simulink model "inverted_pendulum_mpc"  (R2025a)
settings: Solver=ode45  StartTime=0.0  StopTime=30  MaxStep=0.01  RelTol=1e-3
model workspace (MAT data in the model file):
  disturbance_signal = [0  0; 30.1  0]
  mpc_controller = mpc
  mpc_controller.Ts = 0.05
  mpc_controller.PredictionHorizon = 50
  mpc_controller.ControlHorizon = 10
  mpc_controller.Model.Plant = ss
  mpc_controller.Model.Plant.InputName_ = "MV1"
  mpc_controller.Model.Plant.InputGroup_.Manipulated = 1
  mpc_controller.Model.Plant.OutputName_ = ["MO1"; "MO2"; "MO3"; "MO4"]
  mpc_controller.Model.Plant.OutputGroup_.Measured = [1 2 3 4]
  mpc_controller.Model.Plant.IOSize_ = [4 1]
  mpc_controller.Model.Plant.Data_ = ltipack.ssdata
  mpc_controller.Model.Plant.Data_.a = [0  1  0  0; 0  0  -2.4525  0.005; 0  0  0  1; 0  0  12.2625  -0.025]
  mpc_controller.Model.Plant.Data_.b = [0; 0.5; 0; -0.5]
  mpc_controller.Model.Plant.Data_.c = [1  0  0  0; 0  1  0  0; 0  0  1  0; 0  0  0  1]
  mpc_controller.Model.Plant.Data_.d = [0; 0; 0; 0]
  mpc_controller.Model.Plant.Data_.dx0 = [0; 0; 0; 0]
  mpc_controller.Model.Plant.Data_.x0 = [0; 0; 0; 0]
  mpc_controller.Model.Plant.Data_.u0 = 0
  mpc_controller.Model.Plant.Data_.y0 = [0; 0; 0; 0]
  mpc_controller.Model.Plant.Data_.Delay.Input = 0
  mpc_controller.Model.Plant.Data_.Delay.Output = [0; 0; 0; 0]
  mpc_controller.Model.Plant.Data_.Delay.Internal = []
  mpc_controller.Model.Plant.Data_.Ts = 0
  mpc_controller.Model.Disturbance = []
  mpc_controller.Model.Noise = []
  mpc_controller.Model.Nominal.X = [0; 0; 0; 0]
  mpc_controller.Model.Nominal.DX = [0; 0; 0; 0]
  mpc_controller.Model.Nominal.U = 0
  mpc_controller.Model.Nominal.Y = [0; 0; 0; 0]
  mpc_controller.ManipulatedVariables.Min = -10
  mpc_controller.ManipulatedVariables.Max = 10
  mpc_controller.ManipulatedVariables.MinECR = 0
  mpc_controller.ManipulatedVariables.MaxECR = 0
  mpc_controller.ManipulatedVariables.RateMin = -Inf
  mpc_controller.ManipulatedVariables.RateMax = Inf
  mpc_controller.ManipulatedVariables.RateMinECR = 0
  mpc_controller.ManipulatedVariables.RateMaxECR = 0
  mpc_controller.ManipulatedVariables.Target = 'nominal'
  mpc_controller.ManipulatedVariables.Name = 'MV1'
  mpc_controller.ManipulatedVariables.Units = ''
  mpc_controller.ManipulatedVariables.ScaleFactor = 1
  mpc_controller.ManipulatedVariables.Type = 'continuous'
  mpc_controller.OutputVariables(1).Min = -Inf
  mpc_controller.OutputVariables(1).Max = Inf
  mpc_controller.OutputVariables(1).MinECR = 1
  mpc_controller.OutputVariables(1).MaxECR = 1
  mpc_controller.OutputVariables(1).Name = 'MO1'
  mpc_controller.OutputVariables(1).Units = ''
  mpc_controller.OutputVariables(1).ScaleFactor = 1
  mpc_controller.OutputVariables(2).Min = -Inf
  mpc_controller.OutputVariables(2).Max = Inf
  mpc_controller.OutputVariables(2).MinECR = 1
  mpc_controller.OutputVariables(2).MaxECR = 1
  mpc_controller.OutputVariables(2).Name = 'MO2'
  mpc_controller.OutputVariables(2).Units = ''
  mpc_controller.OutputVariables(2).ScaleFactor = 1
  mpc_controller.OutputVariables(3).Min = -Inf
  mpc_controller.OutputVariables(3).Max = Inf
  mpc_controller.OutputVariables(3).MinECR = 1
  mpc_controller.OutputVariables(3).MaxECR = 1
  mpc_controller.OutputVariables(3).Name = 'MO3'
  mpc_controller.OutputVariables(3).Units = ''
  mpc_controller.OutputVariables(3).ScaleFactor = 1
  mpc_controller.OutputVariables(4).Min = -Inf
  mpc_controller.OutputVariables(4).Max = Inf
  mpc_controller.OutputVariables(4).MinECR = 1
  mpc_controller.OutputVariables(4).MaxECR = 1
  mpc_controller.OutputVariables(4).Name = 'MO4'
  mpc_controller.OutputVariables(4).Units = ''
  mpc_controller.OutputVariables(4).ScaleFactor = 1
  mpc_controller.Weights.ManipulatedVariables = 0.707106781187
  mpc_controller.Weights.ManipulatedVariablesRate = 0.1
  mpc_controller.Weights.OutputVariables = [2 1.41421356237 17.3205080757 3.16227766017]
  mpc_controller.Weights.ECR = 100000
  mpc_controller.Optimizer.OptimizationType = 'QP'
  mpc_controller.Optimizer.Solver = 'active-set'
  mpc_controller.Optimizer.SolverOptions = mpc.solver.options.qp.ActiveSet
  mpc_controller.Optimizer.SolverOptions.SolverName = 'ActiveSet'
  mpc_controller.Optimizer.MinOutputECR = 0
  mpc_controller.Optimizer.UseSuboptimalSolution = 0
  mpc_controller.Optimizer.CustomSolver = 0
  mpc_controller.Optimizer.CustomSolverCodeGen = 0
  mpc_controller.History = [2026 11 2 14 24 58.008164]
  mpc_controller.MPCData = mpcdata
  mpc_controller.MPCData.IsDirty = 1
  mpc_controller.MPCData.Ts = 0.05
  mpc_controller.MPCData.p = 50
  mpc_controller.MPCData.m = 10
  mpc_controller.MPCData.UseActiveSetSolver = 1
  mpc_controller.MPCData.UseSuboptimalSolution = 0
  mpc_controller.MPCData.CustomSolver = 0
  mpc_controller.MPCData.CustomSolverCodeGen = 0
  mpc_controller.MPCData.IsCustomEstimation = 1
  mpc_controller.MPCData.Uscale = 1
  mpc_controller.MPCData.Yscale = [1; 1; 1; 1]
  mpc_controller.MPCData.mvindex = 1
  mpc_controller.MPCData.myindex = [1; 2; 3; 4]
  mpc_controller.IsEmpty = 0
  mpc_controller.OldOVIntegrator = {[]; []; []; []}
  mpc_controller.EstGain = 'custom'
  mpc_controller.OutDistModel = ss
  mpc_controller.OutDistModel.IOSize_ = [4 1]
  mpc_controller.OutDistModel.Data_ = ltipack.ssdata
  mpc_controller.OutDistModel.Data_.d = [0; 0; 0; 0]
  mpc_controller.OutDistModel.Data_.u0 = 0
  mpc_controller.OutDistModel.Data_.y0 = [0; 0; 0; 0]
  mpc_controller.OutDistModel.Data_.Delay.Input = 0
  mpc_controller.OutDistModel.Data_.Delay.Output = [0; 0; 0; 0]
  mpc_controller.OutDistModel.Data_.Delay.Internal = []
  mpc_controller.OutDistModel.Data_.Ts = 0
  mpc_controller.Version = '25.1'
libraries: mpclib x1
settings Model: Creator=user  LastModifiedBy=user
settings DataIOCC: SaveOutput=off  SaveTime=off

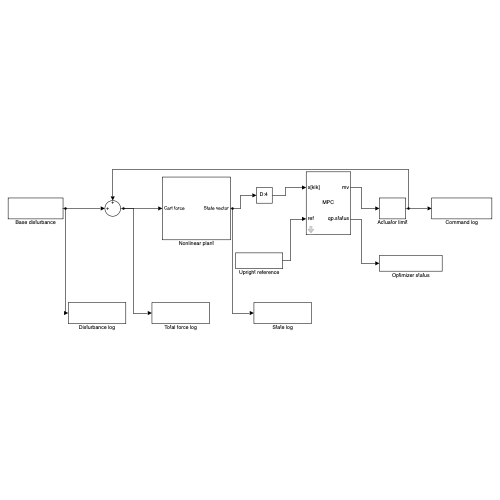
[thumbnail: Simulink's stored preview of the top-level diagram]
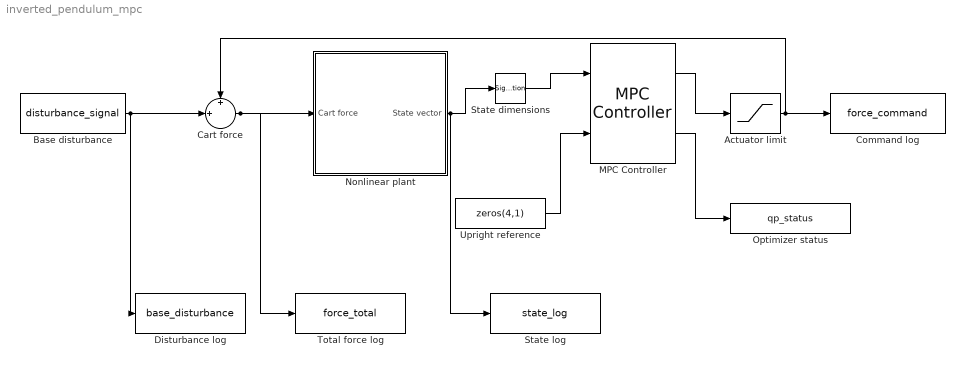
== system inverted_pendulum_mpc ==
  Actuator limit : Saturate  UpperLimit=10  LowerLimit=-10
  Base disturbance : FromWorkspace  VariableName=disturbance_signal  Interpolate=off  OutputAfterFinalValue=Holding final value
  Cart force : Sum  Inputs=+|+||
  Command log : ToWorkspace  VariableName=force_command  SaveFormat=Timeseries  SampleTime=-1
  Disturbance log : ToWorkspace  VariableName=base_disturbance  SaveFormat=Timeseries  SampleTime=-1
  MPC Controller : mpclib/MPC Controller  SCDEnableBlockLinearizationSpecification=on  mpcobj=mpc_controller  is_multiple=0  enable_value=0  return_u0=off  updateMPCinCallerWorkspace=on  md_inport=off  mv_inport=off  uref_inport=off  return_cost=off  return_mvseq=off  return_qpstatus=on  return_xseq=off  return_state=off  return_ovseq=off  state_inport=on  umin_inport=off  umax_inport=off  ymin_inport=off  ymax_inport=off  cc_inport=off  ywt_inport=off  uwt_inport=off  duwt_inport=off  rhoeps_inport=off  pm_inport=off  MaximumP=10  HorizonChoice=FixedHorizon  n_ts=1  n_p=10  n_mv=1  n_md=1  n_ud=0  n_mo=1  n_uo=0  BlockDataType=double  SampleTimeInherited=off  switch_inport=off
  Nonlinear plant : Subsystem
  Optimizer status : ToWorkspace  VariableName=qp_status  SaveFormat=Timeseries  SampleTime=-1
  State dimensions : SignalSpecification  Dimensions=4
  State log : ToWorkspace  VariableName=state_log  SaveFormat=Timeseries  SampleTime=-1
  Total force log : ToWorkspace  VariableName=force_total  SaveFormat=Timeseries  SampleTime=-1
  Upright reference : Constant  Value=zeros(4,1)
  wires:
  Base disturbance/1 -> Cart force/2, Disturbance log/1
  Cart force/1 -> Nonlinear plant/1(Cart force), Total force log/1
  Nonlinear plant/1(State vector) -> State dimensions/1, State log/1
  State dimensions/1 -> MPC Controller/1
  Upright reference/1 -> MPC Controller/2
  MPC Controller/1 -> Actuator limit/1
  MPC Controller/2 -> Optimizer status/1
  Actuator limit/1 -> Cart force/1, Command log/1

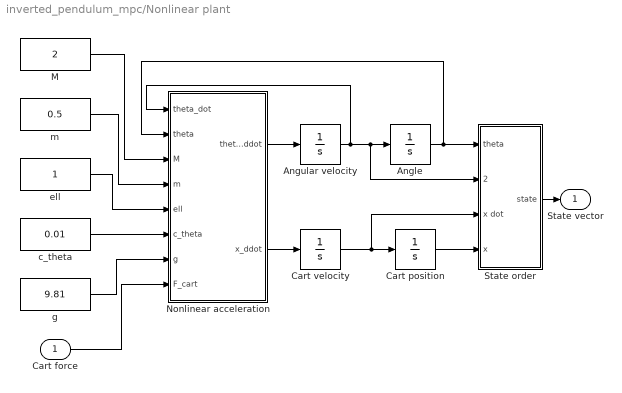
== system inverted_pendulum_mpc/Nonlinear plant ==
  Cart force : Inport
  Angle : Integrator  InitialCondition=5*pi/180
  Angular velocity : Integrator
  Cart position : Integrator
  Cart velocity : Integrator
  M : Constant  Value=2
  Nonlinear acceleration : MATLAB Function  TreatAsAtomicUnit=on
  State order : Subsystem
      mask Display: port_label('input',1,'theta');port_label('input',2,'theta dot');port_label('input',3,'x dot');port_label('input',4,'x');port_label('output',1,'state');
  c_theta : Constant  Value=0.01
  ell : Constant
  g : Constant  Value=9.81
  m : Constant  Value=0.5
  State vector : Outport
  wires:
  M/1 -> Nonlinear acceleration/3(M)
  m/1 -> Nonlinear acceleration/4(m)
  ell/1 -> Nonlinear acceleration/5(ell)
  c_theta/1 -> Nonlinear acceleration/6(c_theta)
  g/1 -> Nonlinear acceleration/7(g)
  Cart force/1 -> Nonlinear acceleration/8(F_cart)
  Nonlinear acceleration/1(theta_ddot) -> Angular velocity/1
  Nonlinear acceleration/2(x_ddot) -> Cart velocity/1
  Angular velocity/1 -> Angle/1, State order/2(theta dot), Nonlinear acceleration/1(theta_dot)
  Cart velocity/1 -> Cart position/1, State order/3(x dot)
  Angle/1 -> Nonlinear acceleration/2(theta), State order/1(theta)
  Cart position/1 -> State order/4(x)
  State order/1(state) -> State vector/1

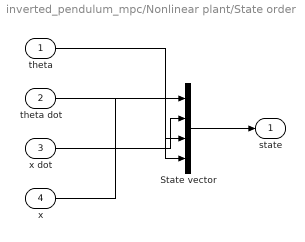
== system inverted_pendulum_mpc/Nonlinear plant/State order ==
  theta : Inport
  theta dot : Inport  Port=2
  x dot : Inport  Port=3
  x : Inport  Port=4
  State vector : Mux
  state : Outport
  wires:
  x/1 -> State vector/1
  x dot/1 -> State vector/2
  theta/1 -> State vector/3
  theta dot/1 -> State vector/4
  State vector/1 -> state/1

== matlab function inverted_pendulum_mpc/Nonlinear plant/Nonlinear acceleration ==
  data: theta_dot input; theta_ddot output; theta input; x_ddot output; M input; m input; ell input; c_theta input; g input; F_cart input
function [theta_ddot, x_ddot] = accelerations(theta_dot, theta, M, m, ell, c_theta, g, F_cart)
% Nonlinear cart-pendulum equations with an applied horizontal cart force.
% Positive theta is the upright perturbation used in Mini Project 1.

s = sin(theta);
c = cos(theta);
mass_matrix = [M + m, m * ell * c; m * ell * c, m * ell^2];
forcing = [F_cart + m * ell * s * theta_dot^2; ...
           m * g * ell * s - c_theta * theta_dot];
acceleration = mass_matrix \ forcing;

x_ddot = acceleration(1);
theta_ddot = acceleration(2);
end
